simulink model "q_current_controller"  (R2025b)
settings: Solver=VariableStepAuto  StartTime=0.0  StopTime=10.0  RelTol=1e-3
undefined symbols (not defined in the file): control
settings Model: Creator=semih  LastModifiedBy=semih
settings GRTTargetCC: CombineOutputUpdateFcns=off

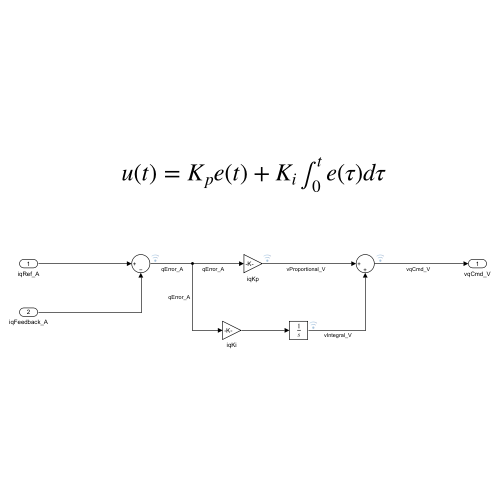
[thumbnail: Simulink's stored preview of the top-level diagram]
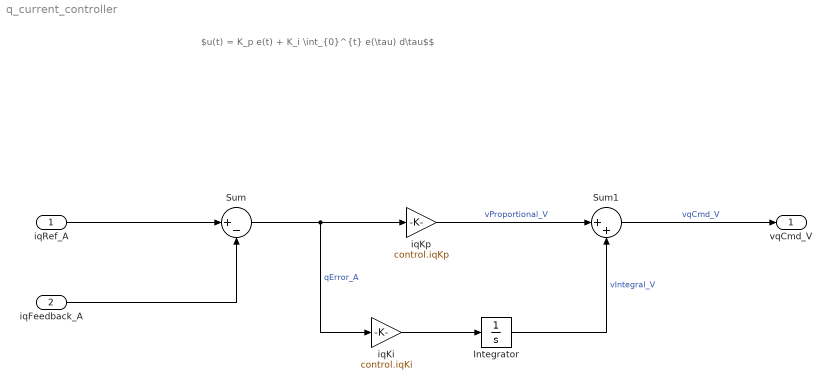
== system q_current_controller ==
  note: $u(t) = K_p e(t) + K_i \int_{0}^{t} e(\tau) d\tau$$
  iqRef_A : Inport
  iqFeedback_A : Inport  Port=2
  Integrator : Integrator
  Sum : Sum  Inputs=|+-
  Sum1 : Sum  Inputs=|++
  iqKi : Gain  Gain=control.iqKi
  iqKp : Gain  Gain=control.iqKp
  vqCmd_V : Outport
  wires:
  iqRef_A/1 -> Sum/1
  iqFeedback_A/1 -> Sum/2
  Sum/1 -> iqKp/1, iqKi/1  "qError_A"
  iqKi/1 -> Integrator/1
  Sum1/1 -> vqCmd_V/1  "vqCmd_V"
  iqKp/1 -> Sum1/1  "vProportional_V"
  Integrator/1 -> Sum1/2  "vIntegral_V"
